simulink model "E6_XYGraph"  (R2024a)
settings: Solver=FixedStepAuto  StartTime=0.0  StopTime=10.0  FixedStep=0.1  RelTol=1e-3
libraries: simulink x1
settings Model: Creator=Sanagostar  LastModifiedBy=Sanagostar

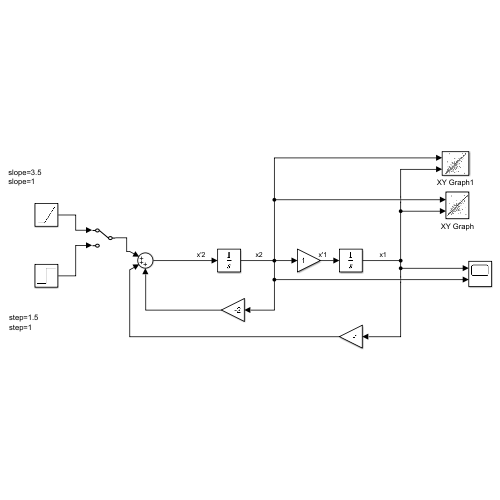
[thumbnail: Simulink's stored preview of the top-level diagram]
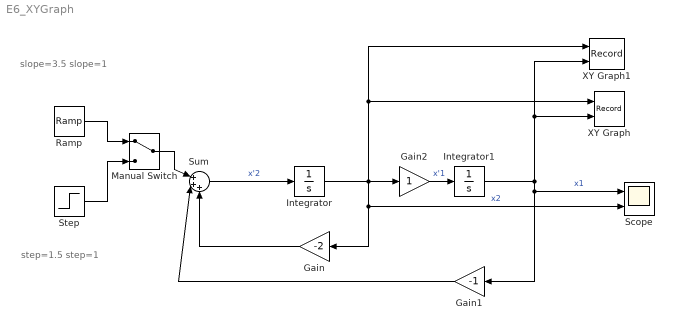
== system E6_XYGraph ==
  note: slope=3.5
      | slope=1
  note: step=1.5
      | step=1
  Gain : Gain  Gain=-2
  Gain1 : Gain  Gain=-1
  Gain2 : Gain
  Integrator : Integrator  InitialCondition=5
  Integrator1 : Integrator  InitialCondition=5
  Manual Switch : ManualSwitch
  Ramp : simulink/Sources/Ramp  slope=3.5  start=0  InitialOutput=0
  Scope : Scope  NumInputPorts=2
  Step : Step  Time=1.5  SampleTime=0
  Sum : Sum  Inputs=|+++
  XY Graph : Record  FileSettingsInternal="{\"entries\":[{\"content\":{\"excelSettings\":{\"content\":{},\"type\":\"Streamout.ExcelSettings\"}},\"type\":\"Streamout.FileSettingStorage\",\"uuid\":\"\"}],\"packageUris\":[\"http:\\/\\/schema.mathworks.com\\/mf0\\/streamout_blocks\\/R2020a\"],\"version\":\"1.0\"}"  Layout=[1 1]  SignalsInternal="{\"entries\":[{\"content\":{},\"type\":\"RecordBlkView.InputSignals\",\"uuid\":\"\"}],\"packageUris\":[\"http:\\/\\/schema.mathworks.com\\/mf0\\/streamout_blocks\\/R2020a\"],\"version\":\"1.0\"}"  VisualizationBindings="{\"xyplotplugin\":{\"info\":[{\"series\":[{\"bindingParametersList\":[{\"parameter\":\"X-Axis\",\"signalID\":287,\"signalName\":\"x2\"},{\"parameter\":\"Y-Axis\",\"signalID\":291,\"signalName\":\"x1\"}],\"seriesID\":0}],\"subplotID\":1}]}}"  CompatibilityTag=XY  st=-1
  XY Graph1 : Record  FileSettingsInternal="{\"entries\":[{\"content\":{\"excelSettings\":{\"content\":{},\"type\":\"Streamout.ExcelSettings\"}},\"type\":\"Streamout.FileSettingStorage\",\"uuid\":\"\"}],\"packageUris\":[\"http:\\/\\/schema.mathworks.com\\/mf0\\/streamout_blocks\\/R2020a\"],\"version\":\"1.0\"}"  Layout=[1 1]  SignalsInternal="{\"entries\":[{\"content\":{\"signals\":[{\"content\":{\"blockPath\":[],\"dimensions\":[1],\"domain\":\"\",\"lineColor\":\"#a2142f\",\"port\":1,\"sid\":[\"\"],\"signalID\":1,\"signalName\":\"x2\"},\"type\":\"RecordBlkView.Signal\",\"uuid\":\"\"},{\"content\":{\"blockPath\":[],\"dimensions\":[1],\"domain\":\"\",\"lineColor\":\"#139fff\",\"port\":2,\"sid\":[\"\"],\"signalID\":2,\"signalName\":\"x1\"},\"type\":\"RecordBlkView.Signal\",\"uuid\":\"\"},{\"content\":{\"blockPath\":[],\"dimensions\":[1],\"domain\":\"\",\"lineColor\":\"#a2142f\",\"plots\":[ 1 ],\"port\":1,\"sid\":[\"\"],\"signalID\":3,\"signalName\":\"x2\"},\"type\":\"RecordBlkView.Signal\",\"uuid\":\"\"},{\"content\":{\"blockPath\":[],\"dimensions\":[1],\"domain\":\"\",\"lineColor\":\"#139fff\",\"plots\":[ 1 ],\"port\":2,\"sid\":[\"\"],\"signalID\":4,\"signalName\":\"x1\"},\"type\":\"RecordBlkView.Signal\",\"uuid\":\"\"}]},\"type\":\"RecordBlkView.InputSignals\",\"uuid\":\"\"}],\"packageUris\":[\"http:\\/\\/schema.mathworks.com\\/mf0\\/streamout_blocks\\/R2020a\"],\"version\":\"1.0\"}"  VisualizationBindings="{\"xyplotplugin\":{\"info\":[{\"series\":[{\"bindingParametersList\":[{\"parameter\":\"X-Axis\",\"signalID\":3,\"signalName\":\"x2\"},{\"parameter\":\"Y-Axis\",\"signalID\":4,\"signalName\":\"x1\"}],\"seriesID\":0}],\"subplotID\":1}]}}"  CompatibilityTag=XY
  wires:
  Gain1/1 -> Sum/2
  Integrator1/1 -> Scope/1, Gain1/1, XY Graph1/2, XY Graph/2  "x1"
  Gain/1 -> Sum/3
  Sum/1 -> Integrator/1  "x'2"
  Integrator/1 -> Gain2/1, Scope/2, Gain/1, XY Graph/1, XY Graph1/1  "x2"
  Ramp/1 -> Manual Switch/1
  Step/1 -> Manual Switch/2
  Manual Switch/1 -> Sum/1
  Gain2/1 -> Integrator1/1  "x'1"
